simulink model "Kinova_Fault_Simulator"  (R2026a)
settings: Solver=ode45  StopTime=5
values from neighbouring files (symbols this model uses):
  x0 = fixed.x0    [solve_flatness_mpc_step_MR.m]
undefined symbols (not defined in the file or in its folder): FaultConfig, Glist_nom, Glist_suc, Mlist_nom, Mlist_suc, Slist_nom, Slist_suc
settings Model: Creator=Johnny  LastModifiedBy=Johnny

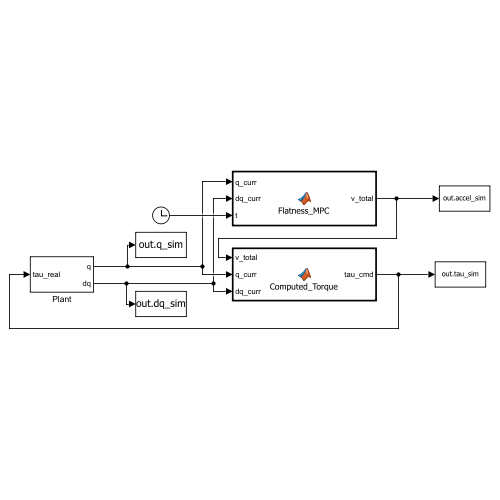
[thumbnail: Simulink's stored preview of the top-level diagram]
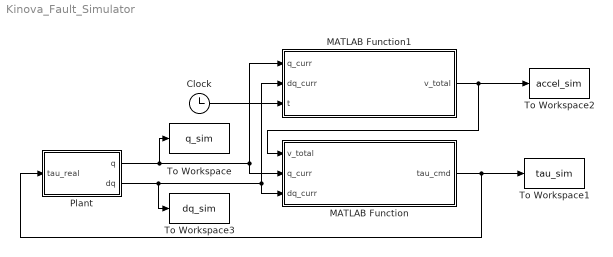
== system Kinova_Fault_Simulator ==
  Clock : Clock
  MATLAB Function : MATLAB Function  TreatAsAtomicUnit=on
  MATLAB Function1 : MATLAB Function  TreatAsAtomicUnit=on
  Plant : Subsystem
  To Workspace : ToWorkspace  VariableName=q_sim  SampleTime=-1
  To Workspace1 : ToWorkspace  VariableName=tau_sim  SampleTime=-1
  To Workspace2 : ToWorkspace  VariableName=accel_sim  SampleTime=-1
  To Workspace3 : ToWorkspace  VariableName=dq_sim  SampleTime=-1
  wires:
  Plant/1(q) -> To Workspace/1, MATLAB Function1/1(q_curr), MATLAB Function/2(q_curr)
  Plant/2(dq) -> To Workspace3/1, MATLAB Function1/2(dq_curr), MATLAB Function/3(dq_curr)
  MATLAB Function1/1(v_total) -> To Workspace2/1, MATLAB Function/1(v_total)
  Clock/1 -> MATLAB Function1/3(t)
  MATLAB Function/1(tau_cmd) -> Plant/1(tau_real), To Workspace1/1

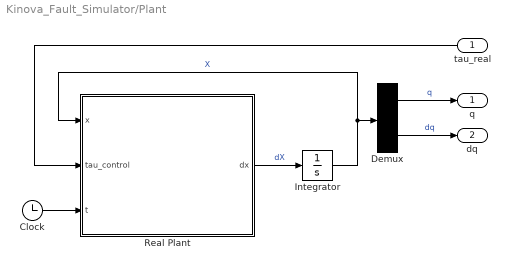
== system Kinova_Fault_Simulator/Plant ==
  tau_real : Inport
  Clock : Clock
  Demux : Demux  Outputs=2
  Integrator : Integrator  InitialCondition=x0
  Real Plant : MATLAB Function  TreatAsAtomicUnit=on
  q : Outport
  dq : Outport  Port=2
  wires:
  tau_real/1 -> Real Plant/2(tau_control)
  Integrator/1 -> Demux/1, Real Plant/1(x)  "X"
  Demux/1 -> q/1  "q"
  Real Plant/1(dx) -> Integrator/1  "dX"
  Demux/2 -> dq/1  "dq"
  Clock/1 -> Real Plant/3(t)

== matlab function Kinova_Fault_Simulator/MATLAB Function ==
  data: v_total input; tau_cmd output; q_curr input; dq_curr input; Mlist_nom parameter; Glist_nom parameter; Slist_nom parameter
function tau_cmd = Computed_Torque(v_total, q_curr, dq_curr, Mlist_nom, Glist_nom, Slist_nom)
% COMPUTED TORQUE (INVERSE DYNAMICS MAPPING)

    % 1. El escudo anti-compilación (si lo necesitas)
    coder.extrinsic('inverse_dynamics_kinova_runtime_MR');
    
    % 2. Creamos la variable y la "bloqueamos" en RAM
    tau_cmd = zeros(6,1); 
    
    % 3. Vectores columna
    q = reshape(q_curr, 6, 1);
    dq = reshape(dq_curr, 6, 1);
    v = reshape(v_total, 6, 1);
    
    % 4. EL TRUCO MÁGICO: Usar (:)
    % Al poner tau_cmd(:), le prohibimos a MATLAB cambiar el tamaño de la variable.
    % Lo obligamos a "rellenar" los 6 espacios que ya creamos.
    tau_cmd(:) = inverse_dynamics_kinova_runtime_MR(q, dq, v, Mlist_nom, Glist_nom, Slist_nom);
end

== matlab function Kinova_Fault_Simulator/Plant/Real Plant ==
  data: x input; dx output; tau_control input; t input; Mlist_suc parameter; Glist_suc parameter; Slist_suc parameter; FaultConfig parameter
function dx = Plant_Dirty(x, tau_control, t, Mlist_suc, Glist_suc, Slist_suc, FaultConfig)
% PLANT_DIRTY: Simulates real physics with parameter uncertainty and wear.
% Calls the state space representation with dirty parameters.
% Uses continuous friction model by passing zero desired acceleration.

    % Llamamos a la función pasándole TODOS los argumentos
    dx = kinova_state_space_sucia_MR(x, tau_control, t, Mlist_suc, Glist_suc, Slist_suc, FaultConfig);
end

== matlab function Kinova_Fault_Simulator/MATLAB Function1 ==
  data: q_curr input; dq_curr input; t input; v_total output; Mlist_nom parameter; Glist_nom parameter; Slist_nom parameter
function v_total = Flatness_MPC(q_curr, dq_curr, t, Mlist_nom, Glist_nom, Slist_nom)
    coder.extrinsic('solve_flatness_mpc_runtime_MR');
    v_total = zeros(6,1);
    v_total(:) = solve_flatness_mpc_runtime_MR(q_curr, dq_curr, t, Mlist_nom, Glist_nom, Slist_nom);
end
